simulink model "sf_tetris2"  (R2025b)
settings: Solver=FixedStepDiscrete  StartTime=0.0  StopTime=inf  FixedStep=1  RelTol=1e-3  EnableMultiTasking=on
CloseFcn:
  | sf_tetris2_gui('close');
settings Model: ExtModeAutoUpdateStatusClock=off  Creator=The MathWorks, Inc.  LastModifiedBy=The MathWorks, Inc.
settings SolverCC: AlgebraicLoopSolver=TrustRegion
settings DataIOCC: LimitDataPoints=on  SaveFormat=Array  ReturnWorkspaceOutputs=off
settings OptimizationCC: ReuseModelBlockBuffer=off  ExpressionDepthLimit=2147483647.0  InitFltsAndDblsToZero=on  EfficientMapNaN2IntZero=off  LifeSpan=inf
settings DebuggingCC: SaveWithParameterizedLinksMsg=none  UnderspecifiedInitializationDetection=Classic  MergeDetectMultiDrivingBlocksExec=none  SignalResolutionControl=TryResolveAllWithWarning  SolverPrmCheckMsg=warning  FcnCallInpInsideContextMsg=warning  UnconnectedInputMsg=warning  UnconnectedOutputMsg=warning  UnconnectedLineMsg=warning  StateNameClashWarn=warning  SFUnexpectedBacktrackingDiag=warning  SFNoUnconditionalDefaultTransitionDiag=warning  SFExecutionAtInitializationDiag=none  ArithmeticOperatorsInVariantConditions=warning
settings HardwareCC: ProdBitPerPointer=32.0  ProdBitPerSizeT=32.0  ProdBitPerPtrDiffT=32.0  ProdLargestAtomicFloat=None  ProdIntDivRoundTo=Undefined  ProdEndianess=Unspecified  ProdWordSize=32.0  ProdHWDeviceType=32-bit Generic
settings ModelReferenceCC: EnableRefExpFcnMdlSchedulingChecks=on  PropagateSignalLabelsOutOfModel=off
settings SFSimCC: SFSimEcho=off  SimUseLocalCustomCode=off  SimParseCustomCode=off  CustomCodeUndefinedFunction=UseInterfaceOnly
settings RTWCC: RTWUseLocalCustomCode=off  GPUComputeCapability=3.5
settings CodeAppCC: StateflowObjectComments=on
settings GRTTargetCC: TargetFcnLib=ansi_tfl_tmw.mat  TargetLangStandard=C89/C90 (ANSI)  CombineOutputUpdateFcns=off  GRTInterface=on
settings ConfigComp: CovMetricSettings=dw  CovSaveCumulativeToWorkspaceVar=on  CovSaveSingleToWorkspaceVar=on  CovExternalEMLEnable=off  CovSFcnEnable=off

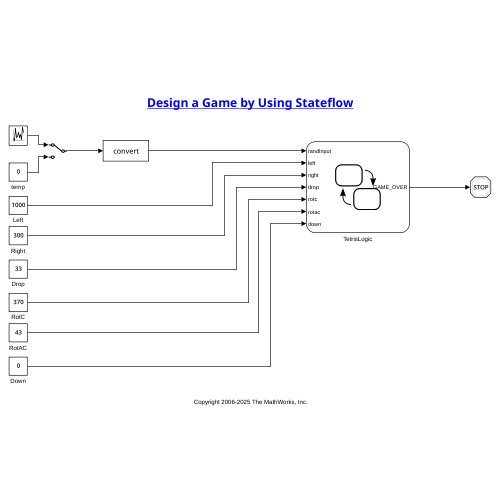
[thumbnail: Simulink's stored preview of the top-level diagram]
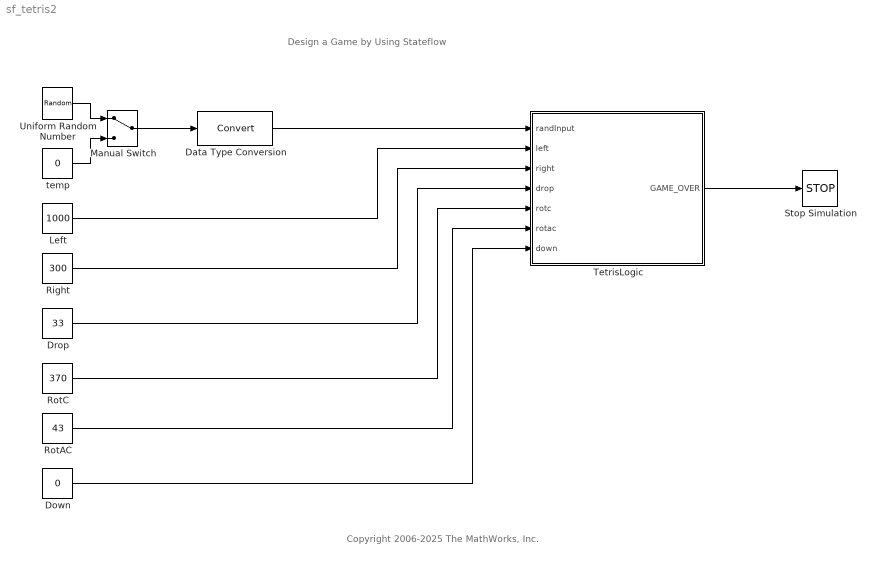
== system sf_tetris2 ==
  note: Copyright 2006-2025 The MathWorks, Inc.
  note: Design a Game by Using Stateflow
  Data Type Conversion : DataTypeConversion  SaturateOnIntegerOverflow=off  RndMeth=Floor
  Down : Constant  Value=0
  Drop : Constant  Value=33
  Left : Constant  Value=1000  OutDataTypeStr=double
  Manual Switch : ManualSwitch
  Right : Constant  Value=300
  RotAC : Constant  Value=43
  RotC : Constant  Value=370
  Stop Simulation : Stop
  TetrisLogic : Stateflow chart  TreatAsAtomicUnit=on
  Uniform Random Number : UniformRandomNumber  Minimum=0  Maximum=7  Seed=20  SampleTime=0
  temp : Constant  Value=0
  wires:
  Data Type Conversion/1 -> TetrisLogic/1(randInput)
  Uniform Random Number/1 -> Manual Switch/1
  temp/1 -> Manual Switch/2
  Manual Switch/1 -> Data Type Conversion/1
  Left/1 -> TetrisLogic/2(left)
  Right/1 -> TetrisLogic/3(right)
  Drop/1 -> TetrisLogic/4(drop)
  RotC/1 -> TetrisLogic/5(rotc)
  RotAC/1 -> TetrisLogic/6(rotac)
  Down/1 -> TetrisLogic/7(down)
  TetrisLogic/1(GAME_OVER) -> Stop Simulation/1

== stateflow chart sf_tetris2/TetrisLogic ==
  state MainArea [parallel]
    settings: executionOrder=2
    state Moving
      state MoveSlowly
        state DOWN [parallel]
          settings: executionOrder=5
          state Down
            en:
            move(0,-1);
          state Idle
            en: counter = 0;
            du: counter++;
          (default) -> Down
          Down -> MainArea.Moving.MoveSlowly.DOWN.Idle
          MainArea.Moving.MoveSlowly.DOWN.Idle -> Down : [after(15-3*level+3,tick)]
        state RIGHT [parallel]
          settings: executionOrder=1
          RIGHT -> (junction 182) : [hasChanged(right)]{move(1,0);}
        state LEFT [parallel]
          settings: executionOrder=2
          LEFT -> (junction 183) : [hasChanged(left)]{move(-1,0);}
        state DOWN_USER [parallel]
          settings: executionOrder=6
          DOWN_USER -> (junction 188) : [hasChanged(down)]{move(0,-1);}
        state ROTAC [parallel]
          settings: executionOrder=3
          ROTAC -> (junction 184) : [hasChanged(rotac)]{shape = rotateAC(shape);}
          (junction 184) -> (junction 185) : [isTouching(px,py)]{shape = rotateC(shape);}
        state ROTC [parallel]
          settings: executionOrder=4
          ROTC -> (junction 186) : [hasChanged(rotc)]{shape = rotateC(shape);}
          (junction 186) -> (junction 187) : [isTouching(px,py)]{shape = rotateAC(shape);}
      state MoveFast
        MoveFast -> (junction 178) : {
            | move(0,-1);
            | dropHeight++;
            | }
      (default) -> MoveSlowly : {dropHeight=0;}
      MoveSlowly -> MoveFast : [hasChanged(drop)]
    state NewShape
      en:
      shape = WaitingArea.shape;
      py = ARENA_HEIGHT;
      px = ARENA_WIDTH/2 + 1;
      send(WaitingArea.NEW);
    state move(dx, dy) [function]
      (default) -> (junction 138) : [!isTouching(px+dx,py+dy)]
          | {
          | px += dx;
          | py += dy;
          | }
    state initArena [function]
      note: Make the "walls" for the arena
      (default) -> (junction 156) : {arena = 0;
          | i = 0;}
      (junction 156) -> (junction 157) [order 1] : [i < ARENA_HEIGHT+1]
      (junction 158) -> (junction 156) : {i++;}
      (junction 156) -> (junction 159) [order 2] : {i = 0;}
      (junction 157) -> (junction 158) : {
          | arena[i][0] = 1;
          | arena[i][ARENA_WIDTH+1] = 1;
          | }
      (junction 159) -> (junction 160) [order 1] : [i < ARENA_WIDTH+2]
      (junction 148) -> (junction 159) : {i++;}
      (junction 159) -> (junction 142) [order 2]
      (junction 160) -> (junction 148) : {
          | arena[0][i] = 1;
          | }
    state NextLevel [group]
      (junction 175) -> (junction 179) : [level < 6]
          | {level++;}
      (junction 181) -> (junction 179) [order 2]
      (junction 181) -> (junction 175) [order 1] : [totalRowsCleared >= 10]
          | {
          | totalRowsCleared = 0;
          | score += 1000*level;
          | initArena();
          | }
    state ist = isTouching(x,y) [function]
      (default) -> (junction 166) : {i=0;}
      (junction 166) -> (junction 143) [order 1] : [i<4]{j=0;}
      (junction 143) -> (junction 141) [order 1] : [j<4]
      (junction 141) -> (junction 139) [order 1] : [y+i >= 0 && y+i < ARENA_HEIGHT+1 ...
          |  && x+j >= 0 && x+j < ARENA_WIDTH+2]
      (junction 143) -> (junction 166) [order 2] : {i++;}
      (junction 166) -> (junction 140) [order 2] : {ist=0;}
      (junction 141) -> (junction 143) [order 2] : {j++;}
      (junction 139) -> (junction 144) : [shape[i][j] && arena[y+i][x+j]]
          | {
          | ist = 1;
          | }
    state freeze [function]
      (default) -> (junction 145) : {i=0;}
      (junction 145) -> (junction 167) [order 1] : [i<4]{j=0;}
      (junction 167) -> (junction 149) [order 1] : [j<4]
      (junction 149) -> (junction 147) [order 1] : [py+i >= 0 && ...
          |  py+i < ARENA_HEIGHT+1 && ...
          |  px+j >= 0 && px+j < ARENA_WIDTH+2]
      (junction 147) -> (junction 146) [order 2]
      (junction 146) -> (junction 167) : {j++;}
      (junction 167) -> (junction 145) [order 2] : {i++;}
      (junction 149) -> (junction 146) [order 2]
      (junction 147) -> (junction 246) [order 1] : [!arena[py+i][px+j] && shape[i][j]]
      (junction 145) -> (junction 150) [order 2]
      (junction 246) -> (junction 146) : {arena[py+i][px+j] = shape[i][j];}
    state Score
      state yesno = isRowMade(r) [function]
        (default) -> (junction 168) : {i = 0;}
        (junction 168) -> (junction 169) [order 1] : [i < ARENA_WIDTH]
        (junction 169) -> (junction 171) [order 1] : [arena[r][i+1]==0]
            | {yesno = 0;}
        (junction 170) -> (junction 168) : {i++;}
        (junction 168) -> (junction 172) [order 2] : {yesno = 1;}
        (junction 169) -> (junction 170) [order 2]
      state clearRow(r) [function]
        (default) -> (junction 173) : {i=r;}
        (junction 173) -> (junction 174) [order 1] : [i < ARENA_HEIGHT]
        (junction 165) -> (junction 173) : {i++;}
        (junction 174) -> (junction 161) : {j=0;}
        (junction 173) -> (junction 164) [order 2]
        (junction 161) -> (junction 162) [order 1] : [j < ARENA_WIDTH]
        (junction 163) -> (junction 161) : {j++;}
        (junction 161) -> (junction 165) [order 2]
        (junction 162) -> (junction 163) : {arena[i][j+1] = ...
            | arena[i+1][j+1];}
      state Done
        en:
        calcScore();
      state ClearCompletedRows
        state Delay
        state Clear
          en:
          clearRow(botRow);
          rowsCleared++;
          totalRowsCleared++;
        (default) -> Clear
        Delay -> Clear : [after(20,tick)]
        Clear -> Delay [order 1] : [isRowMade(botRow)]
      state Tetris
        en:
        // can do some animation
        // here
      (default) -> (junction 180) : {
          | rowsCleared=0;
          | botRow = 1;
          | }
      (junction 177) -> (junction 180) [order 1] : [!isRowMade(botRow)]{botRow++;}
      (junction 180) -> (junction 177) [order 1] : [botRow <= ARENA_HEIGHT]
      (junction 177) -> ClearCompletedRows [order 2] : // botRow is bottom most
          | // fully formed row
      (junction 180) -> Done [order 2] : //no row fully formed
      Clear -> Done [order 3]
      Tetris -> Done : [after(10,tick)]
      Clear -> Tetris [order 2] : [rowsCleared == 4]
    state Stopped
    state FreezeShape
      en:
      freeze();
      shape = 0;
    state GameOver
      en:
      send(GAME_OVER);
    (default) -> NewShape : {initArena();}
    NewShape -> Moving
    Moving -> Stopped : [isTouching(px,py-1)]
    FreezeShape -> Score
    Stopped -> FreezeShape [order 2]
    Stopped -> GameOver [order 1] : [py >= ARENA_HEIGHT]
    (junction 179) -> NewShape
    Done -> (junction 181)
  state WaitingArea [parallel]
    en:
    setShapes();
    settings: executionOrder=1
    state Idle
      en:
      createShapeFrom(randInput);
    state setShapes [function]
      (default) -> (junction 151) : {
          | shapes[0] = 0x00F0;
          | shapes[1] = 0x2260;
          | shapes[2] = 0x4460;
          | shapes[3] = 0x0660;
          | shapes[4] = 0x0360;
          | shapes[5] = 0x0C60;
          | shapes[6] = 0x0270;
          | }
    state createShapeFrom(num) [function]
      (default) -> (junction 152) : {i = 0;}
      (junction 152) -> (junction 153) [order 1] : [i < 16]
      (junction 154) -> (junction 152) : {i++;}
      (junction 152) -> (junction 155) [order 2]
      (junction 153) -> (junction 154) : {
          | r = i/4;
          | c = i%%4;
          | b = (shapes[num] >> i) & 0x0001;
          | shape[r][c] = b*(num+2);
          | }
    WaitingArea.Idle -> WaitingArea.Idle : NEW
  state Draw [parallel]
    en:
    ml.sf_tetris2_gui('init');
    du:
    ml.sf_tetris2_gui('draw', MainArea.arena, MainArea.shape, ...
    WaitingArea.shape, MainArea.px, MainArea.py, ...
    MainArea.score, MainArea.level, MainArea.totalRowsCleared);
    settings: executionOrder=3
  state newShape = rotateAC(shape) [function]
    (default) -> (junction 136) : {
        | newShape[0][0] = shape[3][0];
        | newShape[0][1] = shape[2][0];
        | newShape[0][2] = shape[1][0];
        | newShape[0][3] = shape[0][0];
        |
        | newShape[1][0] = shape[3][1];
        | newShape[1][1] = shape[2][1];
        | newShape[1][2] = shape[1][1];
        | newShape[1][3] = shape[0][1];
        |
        | newShape[2][0] = shape[3][2];
        | newShape[2][1] = shape[2][2];
        | newShape[2][2] = shape[1][2];
        | newShape[2][3] = shape[0][2];
        |
        | newShape[3][0] = shape[3][3];
        | newShape[3][1] = shape[2][3];
        | newShape[3][2] = shape[1][3];
        | newShape[3][3] = shape[0][3];
        | }
  state newShape = rotateC(shape) [function]
    (default) -> (junction 137) : {
        | newShape[0][0] = shape[0][3];
        | newShape[0][1] = shape[1][3];
        | newShape[0][2] = shape[2][3];
        | newShape[0][3] = shape[3][3];
        |
        | newShape[1][0] = shape[0][2];
        | newShape[1][1] = shape[1][2];
        | newShape[1][2] = shape[2][2];
        | newShape[1][3] = shape[3][2];
        |
        | newShape[2][0] = shape[0][1];
        | newShape[2][1] = shape[1][1];
        | newShape[2][2] = shape[2][1];
        | newShape[2][3] = shape[3][1];
        |
        | newShape[3][0] = shape[0][0];
        | newShape[3][1] = shape[1][0];
        | newShape[3][2] = shape[2][0];
        | newShape[3][3] = shape[3][0];
        | }
  data: counter local double; dx function_input int8; dy function_input int8; i temporary uint8; x function_input int8; y function_input int8; ist function_output int8; i temporary int8; j temporary int8; i temporary int8; j temporary int8; yesno function_output double; i temporary int8; r function_input int8; i temporary int8; j temporary int8; r function_input double; rowsCleared local int8; botRow local int8; arena local uint8 size=[ARENA_HEIGHT+1, ARENA_WIDTH+2]; px local int8; py local int8; dropHeight local double; shape local uint8 size=[4,4]; level local uint8 =1; totalRowsCleared local int32; score local double; num function_input uint16; r temporary uint8; c temporary uint8; b temporary uint8; i temporary uint8; shapes local uint16 size=7; shape local uint8 size=[4,4]; shape function_input uint8 size=[4,4]; newShape function_output uint8 size=[4,4]; shape function_input uint8 size=[4,4]; newShape function_output uint8 size=[4,4]; randInput input double; left input double; right input double; drop input double; rotc input double; rotac input double; down input double; ARENA_HEIGHT constant double =20; ARENA_WIDTH constant double =10
  events: NEW local EITHER_EDGE_EVENT; GAME_OVER output EITHER_EDGE_EVENT
  function calcScore:
    | function calcScore
    | % increments the score according to the number of rows currently cleared
    | 
    | persistent linesToScoreMap
    | if isempty(linesToScoreMap)
    |     linesToScoreMap = [40, 100, 300, 1200];
    | end
    | 
    | if rowsCleared > 0
    |     score = score + double(linesToScoreMap(rowsCleared)*level);
    | end
    | score = score + double(dropHeight*level*10);
